simulink model "tb_sens_plant"  (R2026b)
settings: Solver=ode3  StopTime=1  FixedStep=Ts.base  EnableMultiTasking=on
model workspace (MAT data in the model file):
  tbs.cloudN = 2
undefined symbols (not defined in the file or in its folder): Ts
libraries: simulink x1
settings Model: Creator=aomar  LastModifiedBy=aomar
settings ConfigSet: Description=Shaddad fixed-step 1 ms ode3, multitasking, explicit rate transitions (arch 7, D58).
settings DataIOCC: SignalLogging=off
settings OptimizationCC: SimCompilerOptimization=on
settings DebuggingCC: AlgebraicLoopMsg=error  ArtificialAlgebraicLoopMsg=error  SingleTaskRateTransMsg=error  StrictBusMsg=ErrorOnBusTreatedAsVector
settings SimscapeCC: SimscapeNominalValues="[{\"value\":\"1\",\"unit\":\"A\"},{\"value\":\"1\",\"unit\":\"bar\"},{\"value\":\"1\",\"unit\":\"cm^2\"},{\"value\":\"1\",\"unit\":\"cm^3/s\"},{\"value\":\"1\",\"unit\":\"kJ/kg\"},{\"value\":\"1\",\"unit\":\"kW\"},{\"value\":\"1\",\"unit\":\"l\"},{\"value\":\"1\",\"unit\":\"N\"},{\"value\":\"1\",\"unit\":\"N*m\"},{\"value\":\"1\",\"unit\":\"V\"},{\"value\":\"0.001\",\"unit\":\"Wb\"}]"  SimscapeNormalizeSystem=off  SimscapeUseEnergyAccounting=off

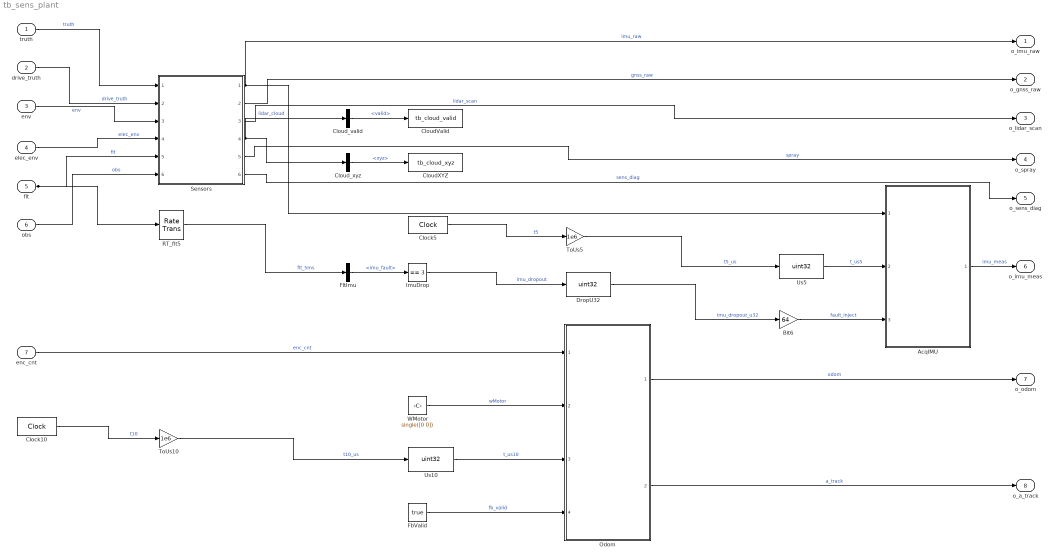
== system tb_sens_plant ==
  truth : Inport  OutDataTypeStr=Bus: Bus_TruthState  SampleTime=Ts.base
  drive_truth : Inport  Port=2  OutDataTypeStr=Bus: Bus_DriveTruth  SampleTime=Ts.base
  env : Inport  Port=3  OutDataTypeStr=Bus: Bus_EnvState  SampleTime=Ts.hk
  elec_env : Inport  Port=4  OutDataTypeStr=Bus: Bus_ElecEnv  SampleTime=Ts.hk
  flt : Inport  Port=5  OutDataTypeStr=Bus: Bus_FaultInject  SampleTime=Ts.ctrl
  obs : Inport  Port=6  OutDataTypeStr=Bus: Bus_ObstaclesDyn  SampleTime=Ts.ctrl
  enc_cnt : Inport  Port=7  OutDataTypeStr=int32  PortDimensions=2  SampleTime=Ts.ctrl
  AcqIMU : Subsystem  ReferencedSubsystem=sens_acq_imu
  Bit6 : Gain  Gain=64  ParamDataTypeStr=uint32  OutDataTypeStr=uint32
  Clock10 : DigitalClock  SampleTime=Ts.ctrl
  Clock5 : DigitalClock  SampleTime=Ts.imu
  CloudValid : ToWorkspace  VariableName=tb_cloud_valid  SaveFormat=Structure With Time  SampleTime=-1
      settings: MaxDataPoints=tbs.cloudN
  CloudXYZ : ToWorkspace  VariableName=tb_cloud_xyz  SaveFormat=Structure With Time  SampleTime=-1
      settings: MaxDataPoints=tbs.cloudN
  Cloud_valid : BusSelector  OutputSignals=valid
  Cloud_xyz : BusSelector  OutputSignals=xyz
  DropU32 : DataTypeConversion  OutDataTypeStr=uint32  SaturateOnIntegerOverflow=off  RndMeth=Floor
  FbValid : Constant  Value=true  OutDataTypeStr=boolean  SampleTime=Ts.ctrl
  FltImu : BusSelector  OutputSignals=imu_fault
  ImuDrop : simulink/Logic and Bit Operations/Compare To Constant  relop===  const=3  OutDataTypeStr=boolean
  Odom : Subsystem  ReferencedSubsystem=sens_odom_compute
  RT_flt5 : RateTransition  OutPortSampleTime=Ts.imu
  Sensors : Subsystem  ReferencedSubsystem=Shaddad_SensorModels
  ToUs10 : Gain  Gain=1e6
  ToUs5 : Gain  Gain=1e6
  Us10 : DataTypeConversion  OutDataTypeStr=uint32  SaturateOnIntegerOverflow=off  RndMeth=Floor
  Us5 : DataTypeConversion  OutDataTypeStr=uint32  SaturateOnIntegerOverflow=off  RndMeth=Floor
  WMotor : Constant  Value=single([0 0])  OutDataTypeStr=single  SampleTime=Ts.ctrl
  o_imu_raw : Outport
  o_gnss_raw : Outport  Port=2
  o_lidar_scan : Outport  Port=3
  o_spray : Outport  Port=4
  o_sens_diag : Outport  Port=5
  o_imu_meas : Outport  Port=6
  o_odom : Outport  Port=7
  o_a_track : Outport  Port=8
  wires:
  truth/1 -> Sensors/1  "truth"
  drive_truth/1 -> Sensors/2  "drive_truth"
  env/1 -> Sensors/3  "env"
  elec_env/1 -> Sensors/4  "elec_env"
  flt/1 -> RT_flt5/1, Sensors/5  "flt"
  obs/1 -> Sensors/6  "obs"
  enc_cnt/1 -> Odom/1  "enc_cnt"
  Clock10/1 -> ToUs10/1  "t10"
  ToUs10/1 -> Us10/1  "t10_us"
  RT_flt5/1 -> FltImu/1  "flt_5ms"
  Sensors/1 -> AcqIMU/1, o_imu_raw/1  "imu_raw"
  Sensors/2 -> o_gnss_raw/1  "gnss_raw"
  Sensors/3 -> o_lidar_scan/1  "lidar_scan"
  Sensors/4 -> Cloud_xyz/1, Cloud_valid/1  "lidar_cloud"
  Sensors/5 -> o_spray/1  "spray"
  Sensors/6 -> o_sens_diag/1  "sens_diag"
  Cloud_valid/1 -> CloudValid/1  "<valid>"
  Cloud_xyz/1 -> CloudXYZ/1  "<xyz>"
  FltImu/1 -> ImuDrop/1  "<imu_fault>"
  ImuDrop/1 -> DropU32/1  "imu_dropout"
  WMotor/1 -> Odom/2  "wMotor"
  FbValid/1 -> Odom/4  "fb_valid"
  Clock5/1 -> ToUs5/1  "t5"
  Us10/1 -> Odom/3  "t_us10"
  ToUs5/1 -> Us5/1  "t5_us"
  DropU32/1 -> Bit6/1  "imu_dropout_u32"
  Odom/1 -> o_odom/1  "odom"
  Odom/2 -> o_a_track/1  "a_track"
  Bit6/1 -> AcqIMU/3  "fault_inject"
  Us5/1 -> AcqIMU/2  "t_us5"
  AcqIMU/1 -> o_imu_meas/1  "imu_meas"
